simulink model "A_ZH_Z1"  (R2026a)
settings: Solver=VariableStepAuto  StopTime=15  MaxStep=500e-3/50
settings Model: Creator=Szalay  LastModifiedBy=Szalay

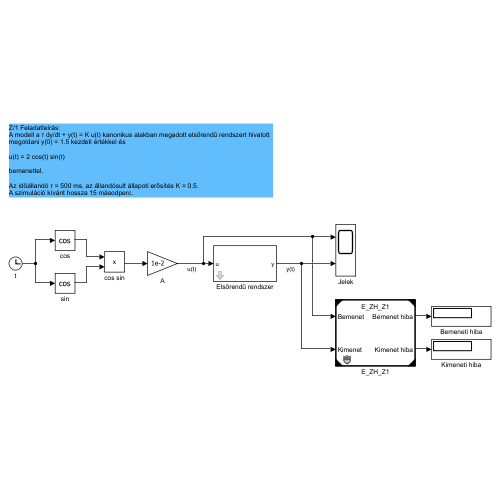
[thumbnail: Simulink's stored preview of the top-level diagram]
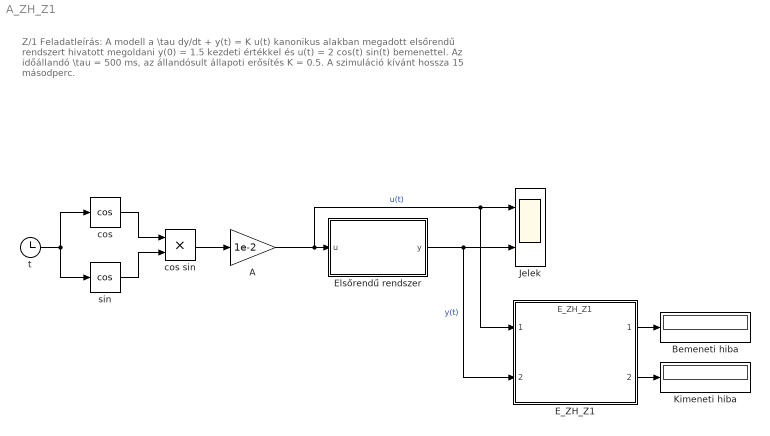
== system A_ZH_Z1 ==
  note: Z/1 Feladatleírás:
      | A modell a \tau dy/dt + y(t) = K u(t) kanonikus alakban megadott elsőrendű rendszert hivatott
      | megoldani y(0) = 1.5 kezdeti értékkel és
      |
      | u(t) = 2 cos(t) sin(t)
      |
      | bemenettel.
      |
      | Az időállandó \tau = 500 ms, az állandósult állapoti erősítés K = 0.5.
      | A szimuláció kívánt hossza 15 másodperc.
  A : Gain  Gain=1e-2
  Bemeneti hiba : Display
  E_ZH_Z1 : ModelReference  ModelNameDialog=E_ZH_Z1.slxp  ModelReferenceVersion=3.0  CopyOfModelProtected=on
  Elsőrendű rendszer : Subsystem  mask(Elsőrendű rendszer){K=0.5, tau=500e-3, y_0=1.5}
      mask prompts: K "Állandósult állapoti erősítés"; tau "Időállandó (s)"; y_0 "A kimenet kezdeti értéke"
      mask help: A lineáris közönséges elsőfokú differenciálegyenlettel jellemzett rendszer modellje.
      mask DialogControl ParameterGroupVar Prompt: Rendszerparaméterek
      mask DialogControl Container3 Prompt: Kezdeti érték
  Jelek : Scope  NumInputPorts=2
      settings: ActiveDisplayYMinimum=-1.3124991345346868  ActiveDisplayYMaximum=1.8124999038371874
  Kimeneti hiba : Display
  cos : Trigonometry  Operator=cos
  cos sin : Product
  sin : Trigonometry  Operator=cos
  t : Clock
  wires:
  t/1 -> cos/1, sin/1
  cos/1 -> cos sin/1
  sin/1 -> cos sin/2
  cos sin/1 -> A/1
  A/1 -> E_ZH_Z1/1, Jelek/1, Elsőrendű rendszer/1(u)  "u(t)"
  E_ZH_Z1/2 -> Kimeneti hiba/1
  Elsőrendű rendszer/1(y) -> E_ZH_Z1/2, Jelek/2  "y(t)"
  E_ZH_Z1/1 -> Bemeneti hiba/1

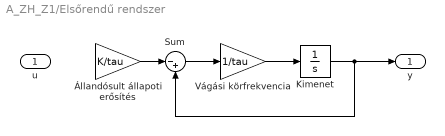
== system A_ZH_Z1/Elsőrendű rendszer ==
  u : Inport
  Kimenet : Integrator  InitialCondition=1.5
  Sum : Sum  Inputs=|-+
  Vágási körfrekvencia : Gain  Gain=1/tau
  Állandósult állapoti erősítés : Gain  Gain=K/tau
  y : Outport
  wires:
  Kimenet/1 -> Sum/2, y/1
  Állandósult állapoti erősítés/1 -> Sum/1
  Vágási körfrekvencia/1 -> Kimenet/1
  Sum/1 -> Vágási körfrekvencia/1
